simulink library "BMS_Library"  (R2025b)
settings: Solver=VariableStepAuto  StartTime=0.0  StopTime=10.0  RelTol=1e-3
undefined symbols (not defined in the file): OCV_empty_V, OCV_full_V, Q_cell_Ah, R0_cell_Ohm, SOC0_module, SOC0_pack, SOC0_plant, Ts
libraries: $bdroot x20
settings Model: Creator=Khadija  LastModifiedBy=Khadija

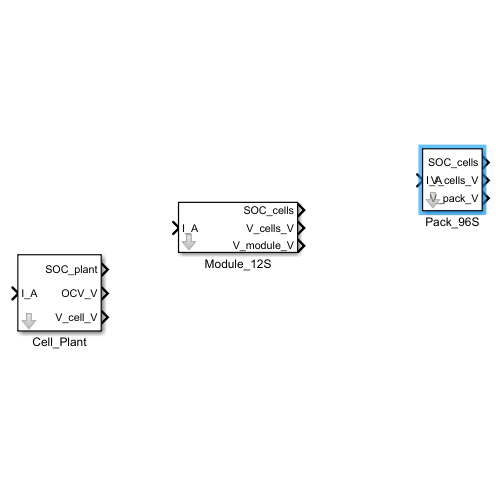
[thumbnail: Simulink's stored preview of the top-level diagram]
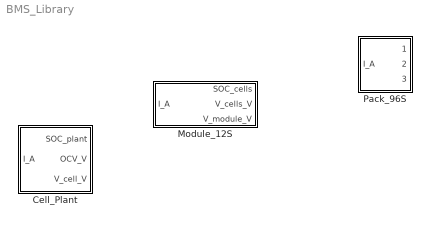
== system BMS_Library ==
  Cell_Plant : Subsystem  mask{SOC_init=SOC0_plant}
      mask prompts: SOC_init "Initial SOC (0 to 1)"
  Module_12S : Subsystem  mask{SOC_init_cells=SOC0_module}
      mask prompts: SOC_init_cells "Initial SOC values (12 cells)"
  Pack_96S : Subsystem  mask{SOC_init_pack=SOC0_pack}
      mask prompts: SOC_init_pack "Initial SOC values (12 cells × 8 modules)"

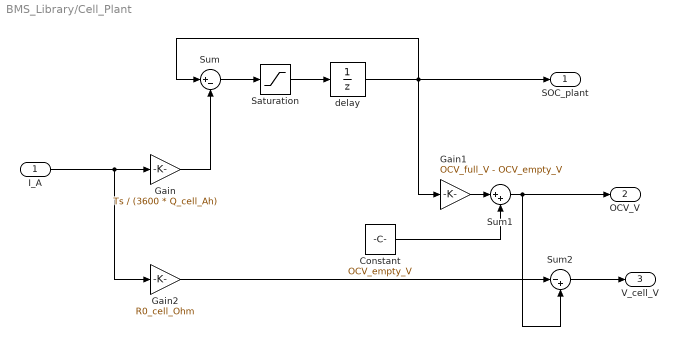
== system BMS_Library/Cell_Plant ==
  I_A : Inport
  Constant : Constant  Value=OCV_empty_V
  Gain : Gain  Gain=Ts / (3600 * Q_cell_Ah)
  Gain1 : Gain  Gain=OCV_full_V - OCV_empty_V
  Gain2 : Gain  Gain=R0_cell_Ohm
  Saturation : Saturate  UpperLimit=1  LowerLimit=0
  Sum : Sum  Inputs=|+-
  Sum1 : Sum  Inputs=|++
  Sum2 : Sum  Inputs=|-+
  delay : UnitDelay  InitialCondition=SOC_init  SampleTime=Ts  HasFrameUpgradeWarning=on
  SOC_plant : Outport
  OCV_V : Outport  Port=2
  V_cell_V : Outport  Port=3
  wires:
  I_A/1 -> Gain2/1, Gain/1
  Gain1/1 -> Sum1/1
  Sum/1 -> Saturation/1
  Sum1/1 -> OCV_V/1, Sum2/2
  Gain/1 -> Sum/2
  Saturation/1 -> delay/1
  Constant/1 -> Sum1/2
  Gain2/1 -> Sum2/1
  Sum2/1 -> V_cell_V/1
  delay/1 -> Gain1/1, Sum/1, SOC_plant/1

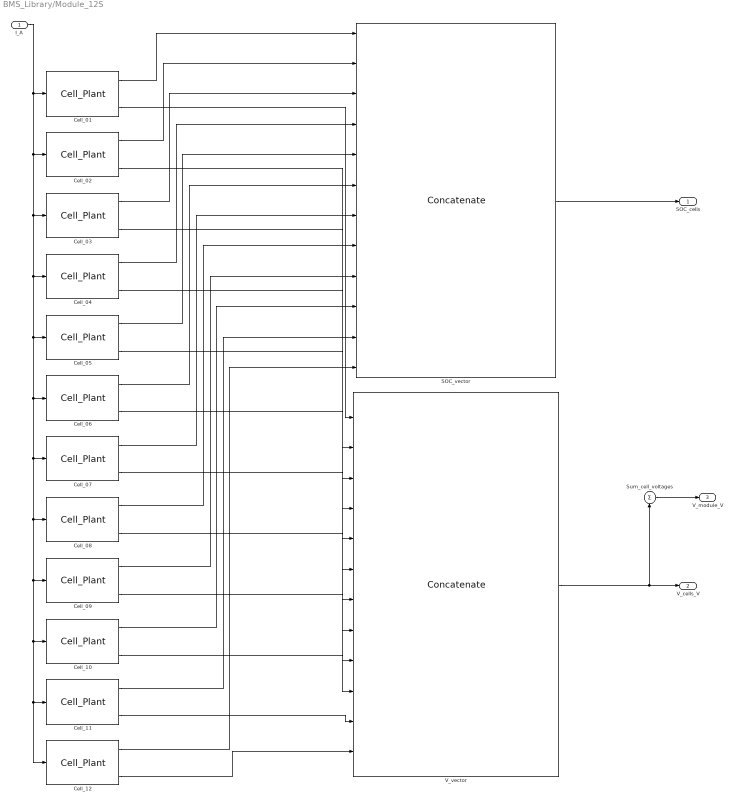
== system BMS_Library/Module_12S ==
  I_A : Inport
  Cell_01 : $bdroot/Cell_Plant  SOC_init=SOC_init_cells(1)
  Cell_02 : $bdroot/Cell_Plant  SOC_init=SOC_init_cells(2)
  Cell_03 : $bdroot/Cell_Plant  SOC_init=SOC_init_cells(3)
  Cell_04 : $bdroot/Cell_Plant  SOC_init=SOC_init_cells(4)
  Cell_05 : $bdroot/Cell_Plant  SOC_init=SOC_init_cells(5)
  Cell_06 : $bdroot/Cell_Plant  SOC_init=SOC_init_cells(6)
  Cell_07 : $bdroot/Cell_Plant  SOC_init=SOC_init_cells(7)
  Cell_08 : $bdroot/Cell_Plant  SOC_init=SOC_init_cells(8)
  Cell_09 : $bdroot/Cell_Plant  SOC_init=SOC_init_cells(9)
  Cell_10 : $bdroot/Cell_Plant  SOC_init=SOC_init_cells(10)
  Cell_11 : $bdroot/Cell_Plant  SOC_init=SOC_init_cells(11)
  Cell_12 : $bdroot/Cell_Plant  SOC_init=SOC_init_cells(12)
  SOC_vector : Concatenate  NumInputs=12
  Sum_cell_voltages : Sum  Inputs=|+
  V_vector : Concatenate  NumInputs=12
  SOC_cells : Outport
  V_cells_V : Outport  Port=2
  V_module_V : Outport  Port=3
  wires:
  I_A/1 -> Cell_11/1, Cell_12/1, Cell_10/1, Cell_09/1, Cell_08/1, Cell_07/1, Cell_06/1, Cell_05/1, Cell_04/1, Cell_03/1, Cell_02/1, Cell_01/1
  Cell_01/1 -> SOC_vector/1
  Cell_02/1 -> SOC_vector/2
  Cell_03/1 -> SOC_vector/3
  Cell_04/1 -> SOC_vector/4
  Cell_05/1 -> SOC_vector/5
  Cell_06/1 -> SOC_vector/6
  Cell_07/1 -> SOC_vector/7
  Cell_08/1 -> SOC_vector/8
  Cell_09/1 -> SOC_vector/9
  Cell_10/1 -> SOC_vector/10
  Cell_11/1 -> SOC_vector/11
  Cell_12/1 -> SOC_vector/12
  SOC_vector/1 -> SOC_cells/1
  Cell_01/3 -> V_vector/1
  Cell_02/3 -> V_vector/2
  Cell_03/3 -> V_vector/3
  Cell_04/3 -> V_vector/4
  Cell_05/3 -> V_vector/5
  Cell_06/3 -> V_vector/6
  Cell_07/3 -> V_vector/7
  Cell_08/3 -> V_vector/8
  Cell_09/3 -> V_vector/9
  Cell_10/3 -> V_vector/10
  Cell_11/3 -> V_vector/11
  Cell_12/3 -> V_vector/12
  V_vector/1 -> Sum_cell_voltages/1, V_cells_V/1
  Sum_cell_voltages/1 -> V_module_V/1

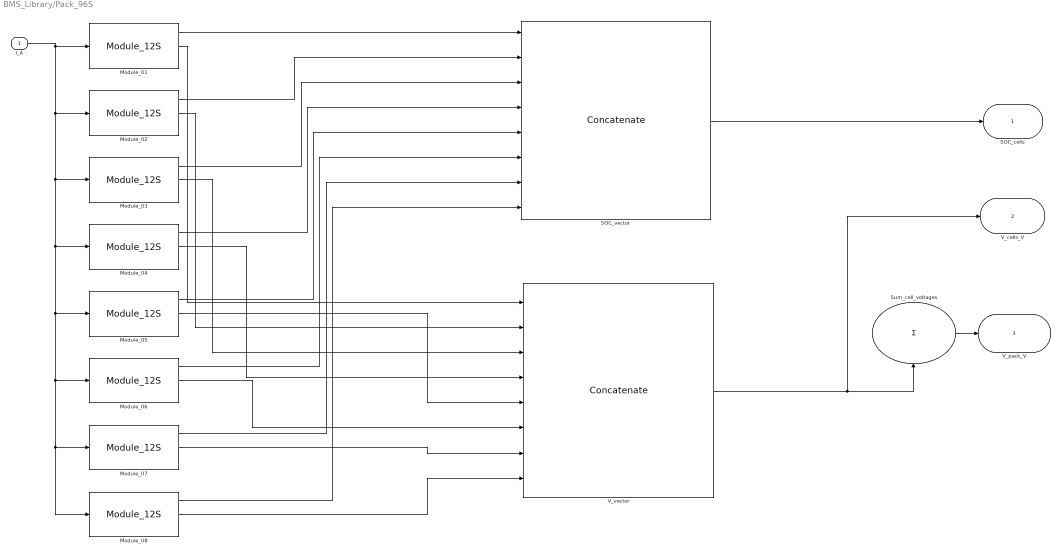
== system BMS_Library/Pack_96S ==
  I_A : Inport
  Module_01 : $bdroot/Module_12S  SOC_init_cells=SOC_init_pack(:, 1)
  Module_02 : $bdroot/Module_12S  SOC_init_cells=SOC_init_pack(:, 2)
  Module_03 : $bdroot/Module_12S  SOC_init_cells=SOC_init_pack(:, 3)
  Module_04 : $bdroot/Module_12S  SOC_init_cells=SOC_init_pack(:, 4)
  Module_05 : $bdroot/Module_12S  SOC_init_cells=SOC_init_pack(:, 5)
  Module_06 : $bdroot/Module_12S  SOC_init_cells=SOC_init_pack(:, 6)
  Module_07 : $bdroot/Module_12S  SOC_init_cells=SOC_init_pack(:, 7)
  Module_08 : $bdroot/Module_12S  SOC_init_cells=SOC_init_pack(:, 8)
  SOC_vector : Concatenate  NumInputs=8
  Sum_cell_voltages : Sum  Inputs=|+
  V_vector : Concatenate  NumInputs=8
  SOC_cells : Outport
  V_cells_V : Outport  Port=2
  V_pack_V : Outport  Port=3
  wires:
  I_A/1 -> Module_07/1, Module_08/1, Module_06/1, Module_05/1, Module_04/1, Module_03/1, Module_02/1, Module_01/1
  Module_01/1 -> SOC_vector/1
  Module_02/1 -> SOC_vector/2
  Module_03/1 -> SOC_vector/3
  Module_04/1 -> SOC_vector/4
  Module_05/1 -> SOC_vector/5
  Module_06/1 -> SOC_vector/6
  Module_07/1 -> SOC_vector/7
  Module_08/1 -> SOC_vector/8
  SOC_vector/1 -> SOC_cells/1
  Module_01/2 -> V_vector/1
  Module_02/2 -> V_vector/2
  Module_03/2 -> V_vector/3
  Module_04/2 -> V_vector/4
  Module_05/2 -> V_vector/5
  Module_06/2 -> V_vector/6
  Module_07/2 -> V_vector/7
  Module_08/2 -> V_vector/8
  V_vector/1 -> V_cells_V/1, Sum_cell_voltages/1
  Sum_cell_voltages/1 -> V_pack_V/1
